simulink model "single_phase_to_three_phase"  (R2026b)
settings: Solver=ode23t  StopTime=0.1  MaxStep=2e-6
libraries: fl_lib x20, nesl_utility x13, ee_lib x3, eePwmGeneratorTwoLevel x1
settings Model: Creator=Arnav  LastModifiedBy=Arnav
settings SimscapeCC: SimscapeLogType=all  SimscapeNominalValues="[{\"value\":\"1\",\"unit\":\"A\"},{\"value\":\"1\",\"unit\":\"bar\"},{\"value\":\"1\",\"unit\":\"cm^2\"},{\"value\":\"1\",\"unit\":\"cm^3/s\"},{\"value\":\"1\",\"unit\":\"kJ/kg\"},{\"value\":\"1\",\"unit\":\"kW\"},{\"value\":\"1\",\"unit\":\"l\"},{\"value\":\"1\",\"unit\":\"N\"},{\"value\":\"1\",\"unit\":\"N*m\"},{\"value\":\"1\",\"unit\":\"V\"},{\"value\":\"0.001\",\"unit\":\"Wb\"}]"  SimscapeUseEnergyAccounting=off

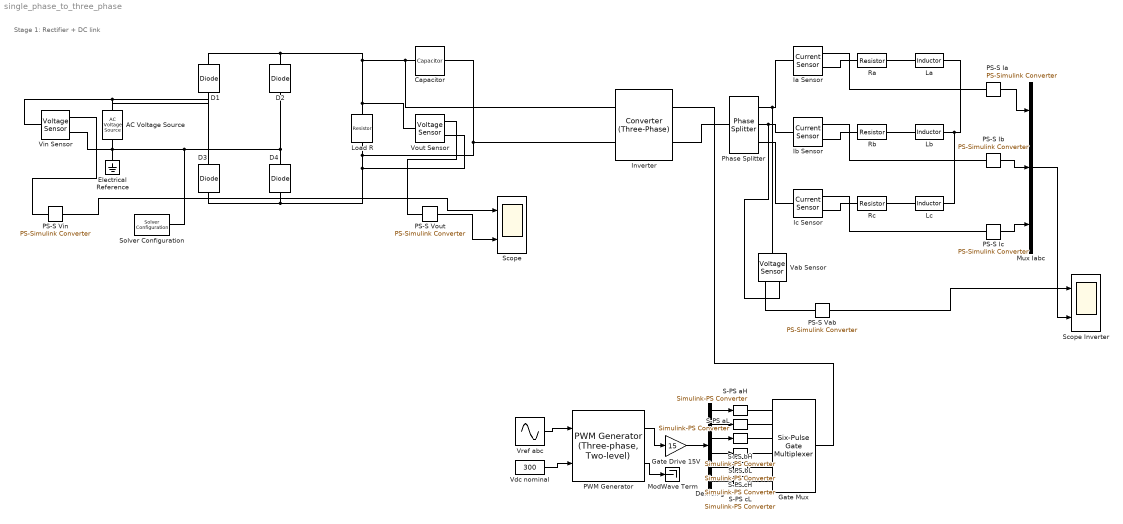
== system single_phase_to_three_phase ==
  note: Stage 1: Rectifier + DC link
  AC Voltage Source : fl_lib/Electrical/Electrical Sources/AC Voltage Source  amp=325 V  shift=0 deg  frequency=50 Hz
  Capacitor : fl_lib/Electrical/Electrical Elements/Capacitor  c=0.0022 F  r=1e-6 Ohm  g=0 1/Ohm  i_specify=off  i_priority=None  i=0 A  i_nominal_specify=off  i_nominal_value=1  i_nominal_unit=A  v_specify=off  v_priority=None  v=0 V  v_nominal_specify=off  v_nominal_value=1  v_nominal_unit=V  vc_specify=off  vc_priority=High  vc=0 V  vc_nominal_specify=off  vc_nominal_value=1  vc_nominal_unit=V
  D{1..4} (4 alike) : fl_lib/Electrical/Electrical Elements/Diode  Vf=0.6 V  Ron=0.3 Ohm  Goff=1e-8 1/Ohm  i_specify=off  i_priority=None  i=0 A  i_nominal_specify=off  i_nominal_value=1  i_nominal_unit=A  v_specify=off  v_priority=None  v=0 V  v_nominal_specify=off  v_nominal_value=1  v_nominal_unit=V
  Demux g : Demux  Outputs=6
  Electrical Reference : fl_lib/Electrical/Electrical Elements/Electrical Reference
  Gate Drive 15V : Gain  Gain=15
  Gate Mux : ee_lib/Semiconductors & Converters/Converters/Six-Pulse Gate Multiplexer  port_option=ee.enum.controlport.ps
  Ia Sensor : fl_lib/Electrical/Electrical Sensors/Current Sensor
  Ib Sensor : fl_lib/Electrical/Electrical Sensors/Current Sensor
  Ic Sensor : fl_lib/Electrical/Electrical Sensors/Current Sensor
  Inverter : ee_lib/Semiconductors & Converters/Converters/Converter (Three-Phase)  port_option=ee.enum.threePhasePort.composite  fidelity_option=ee.enum.converters.fidelity.detailed  device_type=ee.enum.converters.switchingdevice.ideal  showThermalPort=false  K=0  Vth=6 V  Vgt=1 V  Vgt_off=-1 V  Ih=1 A  Vf=0.8 V  Ron=0.001 Ohm  Rds=0.001 Ohm  Goff=1e-6 1/Ohm  Eon_scalar=22.86e-3 J  Eoff_scalar=17.14e-3 J  Eoff_natural_commutation=10e-3 J  Voff=300 V  Iout_scalar=600 A  onCurrentMeasDelay=0 s  useCurrentFromPreviousCycle=false  useVoltageFromPreviousCycle=false  diode_param=ee.enum.converters.protectiondiode.none  diode_Vf=0.8 V  diode_Ron=0.001 Ohm  diode_Goff=1e-5 1/Ohm  diode_C=50 nF  diode_iRM=-235 A  diode_iF=300 A  diode_idot=-50 A/us  diode_trr_param=ee.enum.converters.diodetrr.trr_factor  diode_trr_factor=3  diode_trr=15 us  diode_Qrr=1500 s*uA  diode_rec_loss_model=ee.enum.diode.reverseRecoveryModel.fixed  diode_ErecVal=0 J  diode_scaleWithIandV=false  diode_ErecMat=zeros(2, 3) J  diode_TjrecVec=[298.15, 398.15] K  diode_IfrecVec=[.1, 1, 10] A  diode_IrecVal=10 A  diode_VrecVal=10 V  diode_tFilter=1 / 1000 / 100 s  thermal_network_parameterization=ee.enum.thermalNetworkTopology.external  Rth=[.08, .5] K/W  Rth_Cauer=[.08, .1, .5] K/W  Rth_Foster=[.08, .14, .22, .16] K/W  thermal_mass_parameterization=ee.enum.thermalNetwork.timeconstant  thermal_mass=[.01, .5] J/K  thermal_mass_Cauer=[.01, .1, .5] J/K  thermal_mass_Foster=[.001, .005, .05, .5] J/K  thermal_time_constant=[.001, .2] s  thermal_time_constant_Cauer=[.001, .1, .2] s  thermal_time_constant_Foster=[7e-05, .0007, .01, .08] s  thermal_mass_initial_temperatures=[25, 25] degC  thermal_mass_initial_temperatures_Cauer=[25, 25, 25] degC  junction_thermal_mass=0.01 J/K  Tvec_initial_Foster=[25, 25, 25, 25] degC  snubber_type=ee.enum.converters.snubber.exclude  Cs=1e-7 F  Rs=0.1 Ohm  Vce_loss=[0, 150, 300] V
  La : fl_lib/Electrical/Electrical Elements/Inductor  l=20e-3 H  r=0 Ohm  g=1e-9 1/Ohm  i_specify=off  i_priority=None  i=0 A  i_nominal_specify=off  i_nominal_value=1  i_nominal_unit=A  v_specify=off  v_priority=None  v=0 V  v_nominal_specify=off  v_nominal_value=1  v_nominal_unit=V  i_L_specify=off  i_L_priority=High  i_L=0 A  i_L_nominal_specify=off  i_L_nominal_value=1  i_L_nominal_unit=A
  Lb : fl_lib/Electrical/Electrical Elements/Inductor  l=20e-3 H  r=0 Ohm  g=1e-9 1/Ohm  i_specify=off  i_priority=None  i=0 A  i_nominal_specify=off  i_nominal_value=1  i_nominal_unit=A  v_specify=off  v_priority=None  v=0 V  v_nominal_specify=off  v_nominal_value=1  v_nominal_unit=V  i_L_specify=off  i_L_priority=High  i_L=0 A  i_L_nominal_specify=off  i_L_nominal_value=1  i_L_nominal_unit=A
  Lc : fl_lib/Electrical/Electrical Elements/Inductor  l=20e-3 H  r=0 Ohm  g=1e-9 1/Ohm  i_specify=off  i_priority=None  i=0 A  i_nominal_specify=off  i_nominal_value=1  i_nominal_unit=A  v_specify=off  v_priority=None  v=0 V  v_nominal_specify=off  v_nominal_value=1  v_nominal_unit=V  i_L_specify=off  i_L_priority=High  i_L=0 A  i_L_nominal_specify=off  i_L_nominal_value=1  i_L_nominal_unit=A
  Load R : fl_lib/Electrical/Electrical Elements/Resistor  R=1000 Ohm  i_specify=off  i_priority=None  i=0 A  i_nominal_specify=off  i_nominal_value=1  i_nominal_unit=A  v_specify=off  v_priority=None  v=0 V  v_nominal_specify=off  v_nominal_value=1  v_nominal_unit=V
  ModWave Term : Terminator
  Mux Iabc : Mux  Inputs=3
  PS-S Ia : nesl_utility/PS-Simulink Converter  PhysicalDomain=network_engine_domain  SubClassName=ps_output  LeftPortType=input  RightPortType=output  PseudoPeriodic=off  Frequencies=[]  VectorFormat=inherit  Unit=inherit  AffineConversion=off
  PS-S Ib : nesl_utility/PS-Simulink Converter  PhysicalDomain=network_engine_domain  SubClassName=ps_output  LeftPortType=input  RightPortType=output  PseudoPeriodic=off  Frequencies=[]  VectorFormat=inherit  Unit=inherit  AffineConversion=off
  PS-S Ic : nesl_utility/PS-Simulink Converter  PhysicalDomain=network_engine_domain  SubClassName=ps_output  LeftPortType=input  RightPortType=output  PseudoPeriodic=off  Frequencies=[]  VectorFormat=inherit  Unit=inherit  AffineConversion=off
  PS-S Vab : nesl_utility/PS-Simulink Converter  PhysicalDomain=network_engine_domain  SubClassName=ps_output  LeftPortType=input  RightPortType=output  PseudoPeriodic=off  Frequencies=[]  VectorFormat=inherit  Unit=inherit  AffineConversion=off
  PS-S Vin : nesl_utility/PS-Simulink Converter  PhysicalDomain=network_engine_domain  SubClassName=ps_output  LeftPortType=input  RightPortType=output  PseudoPeriodic=off  Frequencies=[]  VectorFormat=inherit  Unit=inherit  AffineConversion=off
  PS-S Vout : nesl_utility/PS-Simulink Converter  PhysicalDomain=network_engine_domain  SubClassName=ps_output  LeftPortType=input  RightPortType=output  PseudoPeriodic=off  Frequencies=[]  VectorFormat=inherit  Unit=inherit  AffineConversion=off
  PWM Generator : eePwmGeneratorTwoLevel/PWM Generator (Three-phase, Two-level)  PWMMode=Continuous PWM (CPWM)  CPWMMode=SPWM: sinusoidal PWM  DPWMMode=60 DPWM: 60 degree discontinuous PWM  fsw=5e3  Ts=2e-6
      settings: LibrarySourceBlock=|
      | ee_sl_lib/Pulse Width
      | Modulation/PWM Generator
      | (Three-phase, Two-level)
  Phase Splitter : ee_lib/Connectors & References/Phase Splitter
  Ra : fl_lib/Electrical/Electrical Elements/Resistor  R=20 Ohm  i_specify=off  i_priority=None  i=0 A  i_nominal_specify=off  i_nominal_value=1  i_nominal_unit=A  v_specify=off  v_priority=None  v=0 V  v_nominal_specify=off  v_nominal_value=1  v_nominal_unit=V
  Rb : fl_lib/Electrical/Electrical Elements/Resistor  R=20 Ohm  i_specify=off  i_priority=None  i=0 A  i_nominal_specify=off  i_nominal_value=1  i_nominal_unit=A  v_specify=off  v_priority=None  v=0 V  v_nominal_specify=off  v_nominal_value=1  v_nominal_unit=V
  Rc : fl_lib/Electrical/Electrical Elements/Resistor  R=20 Ohm  i_specify=off  i_priority=None  i=0 A  i_nominal_specify=off  i_nominal_value=1  i_nominal_unit=A  v_specify=off  v_priority=None  v=0 V  v_nominal_specify=off  v_nominal_value=1  v_nominal_unit=V
  S-PS aH : nesl_utility/Simulink-PS Converter  PhysicalDomain=network_engine_domain  SubClassName=ps_input  LeftPortType=input  RightPortType=output  PseudoPeriodic=off  Frequencies=[]  NoiseDistribution=none  NoiseParameters=[]  Unit=1  AffineConversion=off  FilteringAndDerivatives=provide  SimscapeFilterOrder=1  InputFilterTimeConstant=0.001  UdotUserProvided=0
  S-PS aL : nesl_utility/Simulink-PS Converter  PhysicalDomain=network_engine_domain  SubClassName=ps_input  LeftPortType=input  RightPortType=output  PseudoPeriodic=off  Frequencies=[]  NoiseDistribution=none  NoiseParameters=[]  Unit=1  AffineConversion=off  FilteringAndDerivatives=provide  SimscapeFilterOrder=1  InputFilterTimeConstant=0.001  UdotUserProvided=0
  S-PS bH : nesl_utility/Simulink-PS Converter  PhysicalDomain=network_engine_domain  SubClassName=ps_input  LeftPortType=input  RightPortType=output  PseudoPeriodic=off  Frequencies=[]  NoiseDistribution=none  NoiseParameters=[]  Unit=1  AffineConversion=off  FilteringAndDerivatives=provide  SimscapeFilterOrder=1  InputFilterTimeConstant=0.001  UdotUserProvided=0
  S-PS bL : nesl_utility/Simulink-PS Converter  PhysicalDomain=network_engine_domain  SubClassName=ps_input  LeftPortType=input  RightPortType=output  PseudoPeriodic=off  Frequencies=[]  NoiseDistribution=none  NoiseParameters=[]  Unit=1  AffineConversion=off  FilteringAndDerivatives=provide  SimscapeFilterOrder=1  InputFilterTimeConstant=0.001  UdotUserProvided=0
  S-PS cH : nesl_utility/Simulink-PS Converter  PhysicalDomain=network_engine_domain  SubClassName=ps_input  LeftPortType=input  RightPortType=output  PseudoPeriodic=off  Frequencies=[]  NoiseDistribution=none  NoiseParameters=[]  Unit=1  AffineConversion=off  FilteringAndDerivatives=provide  SimscapeFilterOrder=1  InputFilterTimeConstant=0.001  UdotUserProvided=0
  S-PS cL : nesl_utility/Simulink-PS Converter  PhysicalDomain=network_engine_domain  SubClassName=ps_input  LeftPortType=input  RightPortType=output  PseudoPeriodic=off  Frequencies=[]  NoiseDistribution=none  NoiseParameters=[]  Unit=1  AffineConversion=off  FilteringAndDerivatives=provide  SimscapeFilterOrder=1  InputFilterTimeConstant=0.001  UdotUserProvided=0
  Scope : Scope  NumInputPorts=2
      settings: ActiveDisplayYMinimum=-406.24650285074631  ActiveDisplayYMaximum=406.24882907551813
  Scope Inverter : Scope  NumInputPorts=2
      settings: ActiveDisplayYMinimum=-391.49280790520226  ActiveDisplayYMaximum=391.51312367371412
  Solver Configuration : nesl_utility/Solver Configuration  PhysicalDomain=network_engine_domain  SubClassName=solver  LeftPortType=input  RightPortType=generic  Tones=[]  Harmonics=[]  SimulateNoise=off  Profile=off  UseLocalSampling=off  EnableSwitchedLinearOptims=on  FrequencyDomain=off  UseCCode=off  RelTol=0.001  AbsTol=0.001  MinStep=1e-09  ToWorkspace=off  RevertToSquareIcSolve=off  NumHomotopyIterations=100  PhasorMode=off  PhasorModeNumHarmonics=1  ConsistencySolver=NEWTON_XTOL_AFTER_FTOL  CanonicalOrdering=CANONICAL  OptimizeIntermediates=OPTIMIZED  MulticoreSolverChoice=BACKWARD_EULER  IndexReductionMethod=DerivativeReplacement  DoDC=off  ResidualTolerance=1e-09  ConsistencyTolSource=GLOBAL  ConsistencyAbsTol=0.001  ConsistencyRelTol=0.001  ConsistencyTolFactor=0.001  UseLocalSolver=off  LocalSolverChoice=NE_BACKWARD_EULER_ADVANCER  ResolveIndetEquations=on  FunctionEvalNumThread=1  LocalSolverSampleTime=0.001  DoFixedCost=off  MaxNonlinIter=3  MaxModeIter=2  ComputeImpulses=off  ImpulseIterations=2  LinearAlgebra=auto  LinearAlgebraNumThread=0  EquationFormulation=NE_TIME_EF  DelaysMemoryBudget=1024  AutomaticFiltering=on  FilteringTimeConstant=0.001  PartitionStorageMethod=AS_NEEDED  PartitionMemoryBudget=1024  PartitionMethod=BALANCED  MultibodyUseLocalSolver=off  MultibodyLocalSolverChoice=ODE1  MultibodyLocalSolverSampleTime=0.001
  Vab Sensor : fl_lib/Electrical/Electrical Sensors/Voltage Sensor
  Vdc nominal : Constant  Value=300
  Vin Sensor : fl_lib/Electrical/Electrical Sensors/Voltage Sensor
  Vout Sensor : fl_lib/Electrical/Electrical Sensors/Voltage Sensor
  Vref abc : Sin  Amplitude=120  Frequency=2*pi*50  Phase=[0 -2*pi/3 2*pi/3]  SampleTime=0
  wires:
  PS-S Vin/1 -> Scope/1
  PS-S Vout/1 -> Scope/2
  PS-S Ia/1 -> Mux Iabc/1
  PS-S Ib/1 -> Mux Iabc/2
  PS-S Ic/1 -> Mux Iabc/3
  PS-S Vab/1 -> Scope Inverter/1
  Mux Iabc/1 -> Scope Inverter/2
  Vref abc/1 -> PWM Generator/1
  Vdc nominal/1 -> PWM Generator/2
  PWM Generator/2 -> ModWave Term/1
  PWM Generator/1 -> Gate Drive 15V/1
  Gate Drive 15V/1 -> Demux g/1
  Demux g/1 -> S-PS aH/1
  Demux g/2 -> S-PS aL/1
  Demux g/3 -> S-PS bH/1
  Demux g/4 -> S-PS bL/1
  Demux g/5 -> S-PS cH/1
  Demux g/6 -> S-PS cL/1
  connections:
  D2/RConn1 -- D1/RConn1 -- Vout Sensor/LConn1 -- Load R/LConn1 -- Capacitor/LConn1 -- Inverter/RConn1
  D4/LConn1 -- D3/LConn1 -- Capacitor/RConn1 -- Inverter/RConn2 -- Load R/RConn1 -- Vout Sensor/RConn2
  Electrical Reference/LConn1 -- Solver Configuration/RConn1 -- D4/RConn1 -- D2/LConn1 -- AC Voltage Source/RConn1 -- Vin Sensor/RConn2
  D1/LConn1 -- AC Voltage Source/LConn1 -- D3/RConn1 -- Vin Sensor/LConn1
  Vin Sensor/RConn1 -- PS-S Vin/LConn1
  Vout Sensor/RConn1 -- PS-S Vout/LConn1
  Inverter/LConn2 -- Phase Splitter/LConn1
  Ia Sensor/LConn1 -- Phase Splitter/RConn1 -- Vab Sensor/LConn1
  Ia Sensor/RConn2 -- Ra/LConn1
  Ra/RConn1 -- La/LConn1
  Ia Sensor/RConn1 -- PS-S Ia/LConn1
  Ib Sensor/LConn1 -- Phase Splitter/RConn2 -- Vab Sensor/RConn2
  Ib Sensor/RConn2 -- Rb/LConn1
  Rb/RConn1 -- Lb/LConn1
  Ib Sensor/RConn1 -- PS-S Ib/LConn1
  Phase Splitter/RConn3 -- Ic Sensor/LConn1
  Ic Sensor/RConn2 -- Rc/LConn1
  Rc/RConn1 -- Lc/LConn1
  Ic Sensor/RConn1 -- PS-S Ic/LConn1
  Lb/RConn1 -- La/RConn1 -- Lc/RConn1
  Vab Sensor/RConn1 -- PS-S Vab/LConn1
  S-PS aH/RConn1 -- Gate Mux/LConn1
  S-PS aL/RConn1 -- Gate Mux/LConn2
  S-PS bH/RConn1 -- Gate Mux/LConn3
  S-PS bL/RConn1 -- Gate Mux/LConn4
  S-PS cH/RConn1 -- Gate Mux/LConn5
  S-PS cL/RConn1 -- Gate Mux/LConn6
  Gate Mux/RConn1 -- Inverter/LConn1
